simulink model "turbo_controller"  (R2025a)
settings: Solver=FixedStepAuto  StartTime=0.0  StopTime=inf  FixedStep=0.001  RelTol=1e-3
PostLoadFcn:
  | % 自动定位同目录CubeMX文件；不需要外部初始化脚本。
  | codertarget.data.setParameterValue('turbo_controller','STM32CubeMX.ProjectFile',fullfile(fileparts(get_param('turbo_controller','FileName')),'turbo_f407.ioc'));
InitFcn:
  | % 中文说明：按原控制器字段与类型创建三组接口总线；控制参数已内嵌。
  | tc_names=["EValve_Cycle" "EValve_Open" "Eblast_Cycle" "Eblast_Open" "Motor_Cycle" "Motor_Open" "EValve_Enable" "Eblast_Enable" "Motor_Enable" "SWO_Firework" "SWO_BleedAir" "EngineState" "Flag_ECUReset_Clear" "Flag_ECUReset_Save" "Flag_Reset_Enable" "Accelerator" "Nc_dem" "Nc"]; tc_types=["uint16" "uint16" "uint16" "uint16" "uint16" "uint16" "uint8" "uint8" "uint8" "uint8" "uint8" "uint8" "uint8" "uint8" "uint8" "single" "single" "single"];
  | for tc_k=1:numel(tc_names)
  |  tc_e(tc_k)=Simulink.BusElement; tc_e(tc_k).Name=char(tc_names(tc_k)); tc_e(tc_k).DataType=char(tc_types(tc_k));
  | end
  | EngineControl_Out=Simulink.Bus; EngineControl_Out.DataScope='Exported'; EngineControl_Out.Elements=tc_e;
  | clear tc_e tc_names tc_types tc_k
  | tc_names=["savedata1" "savedata2" "savedata3" "savedata4" "savedata5" "savedata6" "savedata7" "savedata8" "savedata9" "savedata10" "savedata11" "savedata12" "savedata13" "savedata14" "savedata15" "savedata16" "savedata17" "savedata18" "savedata19" "savedata20" "savedata21" "savedata22" "savedata23" "savedata24" "savedata25"]; tc_types=["single" "single" "single" "single" "single" "single" "single" "single" "single" "single" "single" "single" "single" "single" "single" "single" "single" "single" "single" "single" "single" "single" "single" "single" "single"];
  | for tc_k=1:numel(tc_names)
  |  tc_e(tc_k)=Simulink.BusElement; tc_e(tc_k).Name=char(tc_names(tc_k)); tc_e(tc_k).DataType=char(tc_types(tc_k));
  | end
  | SaveData_Out=Simulink.Bus; SaveData_Out.DataScope='Exported'; SaveData_Out.Elements=tc_e;
  | clear tc_e tc_names tc_types tc_k
  | tc_names=["senddata1" "senddata2" "senddata3" "senddata4" "senddata5" "senddata6" "senddata7" "senddata8" "senddata9" "senddata10" "senddata11" "senddata12" "senddata13" "senddata14" "senddata15" "senddata16" "senddata17" "senddata18" "senddata19" "senddata20" "senddata21" "senddata22" "senddata23" "senddata24" "senddata25" "senddata26" "senddata27" "senddata28" "senddata29"]; tc_types=["uint8" "uint8" "uint8" "uint8" "uint8" "uint8" "uint8" "uint8" "uint8" "uint8" "uint8" "uint8" "uint8" "uint8" "uint8" "uint8" "uint8" "uint8" "uint8" "uint8" "uint8" "uint8" "uint8" "uint8" "uint8" "uint8" "uint8" "uint8" "uint8"];
  | for tc_k=1:numel(tc_names)
  |  tc_e(tc_k)=Simulink.BusElement; tc_e(tc_k).Name=char(tc_names(tc_k)); tc_e(tc_k).DataType=char(tc_types(tc_k));
  | end
  | SendData_Out=Simulink.Bus; SendData_Out.DataScope='Exported'; SendData_Out.Elements=tc_e;
  | clear tc_e tc_names tc_types tc_k
  | 
  | % 以下为接口中文说明；只设置描述，不改变数值或数据类型。
  | EngineControl_Out.Description='执行控制输出（阀、电机、点火、状态及复位请求）';
  | tc_cn=["EValve_Cycle（主油阀周期计数（每计数2毫秒））" "EValve_Open（主油阀开通计数（每计数2毫秒））" "Eblast_Cycle（副油阀周期计数（每计数2毫秒））" "Eblast_Open（副油阀开通计数（每计数2毫秒））" "Motor_Cycle（起动电机周期计数）" "Motor_Open（起动电机开通计数）" "EValve_Enable（主油阀驱动使能）" "Eblast_Enable（副油阀驱动使能）" "Motor_Enable（起动电机使能）" "SWO_Firework（点火器使能（1开））" "SWO_BleedAir（引气阀使能（1开））" "EngineState（发动机状态）" "Flag_ECUReset_Clear（清除复位恢复状态请求）" "Flag_ECUReset_Save（保存复位恢复数据请求）" "Flag_Reset_Enable（处理器软件复位请求）" "Accelerator（油门／油泵给定控制量）" "Nc_dem（控制目标转速）" "Nc（发动机反馈转速（转每分））"];
  | tc_elements=EngineControl_Out.Elements;
  | for tc_k=1:numel(tc_cn)
  |  tc_elements(tc_k).Description=char(tc_cn(tc_k));
  | end
  | EngineControl_Out.Elements=tc_elements;
  | clear tc_cn tc_elements tc_k
  | SaveData_Out.Description='25项运行记录；字段含义按当前模型数据来源解释';
  | tc_cn=["savedata1（指令回显记录）" "savedata2（入口总温记录（℃））" "savedata3（电源电压记录）" "savedata4（排气温度记录（℃））" "savedata5（标定燃油压力记录）" "savedata6（副油阀占空比记录（％））" "savedata7（主油阀占空比记录（％））" "savedata8（温度修正转速记录）" "savedata9（开关输出及反馈位域）" "savedata10（物理转速记录）" "savedata11（油泵目标给定原始值）" "savedata12（起动电机占空比记录（％））" "savedata13（发动机状态码记录）" "savedata14（故障告警位域记录）" "savedata15（模型记录帧序号）" "savedata16（处理器温度记录（℃））" "savedata17（装订转速记录（沿用旧电源字段名））" "savedata18（导航高度记录）" "savedata19（飞行空速记录）" "savedata20（主阀旧记录位（恒零保留））" "savedata21（第21项保留记录（恒零））" "savedata22（保留记录项22）" "savedata23（保留记录项23）" "savedata24（保留记录项24）" "savedata25（保留记录项25）"];
  | tc_elements=SaveData_Out.Elements;
  | for tc_k=1:numel(tc_cn)
  |  tc_elements(tc_k).Description=char(tc_cn(tc_k));
  | end
  | SaveData_Out.Elements=tc_elements;
  | clear tc_cn tc_elements tc_k
  | SendData_Out.Description='29字段回传及外设命令接口；板端上位机帧只取第3至27字段';
  | tc_cn=["senddata1（回传发送允许标志（不直接上线路））" "senddata2（回传载荷长度25字节）" "senddata3（回传指令回显字节）" "senddata4（总温编码字节（℃＋80））" "senddata5（电源电压编码字节）" "senddata6（排温编码高字节）" "senddata7（排温编码低字节）" "senddata8（燃油压力编码高字节）" "senddata9（燃油压力编码低字节）" "senddata10（副油阀占空比字节（％））" "senddata11（主油阀占空比字节（％））" "senddata12（修正转速编码高字节）" "senddata13（修正转速编码低字节）" "senddata14（驱动及反馈状态位域）" "senddata15（物理转速编码高字节）" "senddata16（物理转速编码低字节）" "senddata17（油泵目标给定高字节（串口二使用））" "senddata18（油泵目标给定低字节（串口二使用））" "senddata19（起动电机占空比命令（串口一使用））" "senddata20（发动机状态码字节）" "senddata21（故障告警位域字节）" "senddata22（帧序号占位（板端另行填写））" "senddata23（处理器温度编码（℃＋50））" "senddata24（控制目标转速编码高字节）" "senddata25（控制目标转速编码低字节）" "senddata26（占位字节（板端改填实测泵速高字节））" "senddata27（占位字节（板端改填实测泵速低字节））" "senddata28（装订转速高字节（本板未发送））" "senddata29（装订转速低字节（本板未发送））"];
  | tc_elements=SendData_Out.Elements;
  | for tc_k=1:numel(tc_cn)
  |  tc_elements(tc_k).Description=char(tc_cn(tc_k));
  | end
  | SendData_Out.Elements=tc_elements;
  | clear tc_cn tc_elements tc_k
  | 
  | 
  | % FRAM模块化事务：接口类型和上电初始状态，随模型保存，无外部初始化文件。
  | clear FM_elements
  | FM_elements(1)=Simulink.BusElement;FM_elements(1).Name='phase';FM_elements(1).DataType='uint8';FM_elements(1).Dimensions=[1 1];FM_elements(1).Description='phase（当前事务阶段）';
  | FM_elements(2)=Simulink.BusElement;FM_elements(2).Name='a';FM_elements(2).DataType='uint8';FM_elements(2).Dimensions=[64 1];FM_elements(2).Description='a（启动时缓存的首区64字节）';
  | FM_elements(3)=Simulink.BusElement;FM_elements(3).Name='active';FM_elements(3).DataType='uint16';FM_elements(3).Dimensions=[1 1];FM_elements(3).Description='active（当前有效记录区地址）';
  | FM_elements(4)=Simulink.BusElement;FM_elements(4).Name='generation';FM_elements(4).DataType='uint32';FM_elements(4).Dimensions=[1 1];FM_elements(4).Description='generation（当前有效记录代号）';
  | FM_elements(5)=Simulink.BusElement;FM_elements(5).Name='record';FM_elements(5).DataType='uint8';FM_elements(5).Dimensions=[64 1];FM_elements(5).Description='record（本次冻结的待写记录）';
  | FM_elements(6)=Simulink.BusElement;FM_elements(6).Name='addr';FM_elements(6).DataType='uint16';FM_elements(6).Dimensions=[1 1];FM_elements(6).Description='addr（本次备用写入地址）';
  | FM_elements(7)=Simulink.BusElement;FM_elements(7).Name='lastSave';FM_elements(7).DataType='single';FM_elements(7).Dimensions=[1 1];FM_elements(7).Description='lastSave（上次开始保存的秒数）';
  | FM_elements(8)=Simulink.BusElement;FM_elements(8).Name='lastState';FM_elements(8).DataType='uint8';FM_elements(8).Dimensions=[1 1];FM_elements(8).Description='lastState（上次保存时的发动机状态）';
  | FM_elements(9)=Simulink.BusElement;FM_elements(9).Name='boot';FM_elements(9).DataType='boolean';FM_elements(9).Dimensions=[1 1];FM_elements(9).Description='boot（启动记录是否允许恢复）';
  | FM_elements(10)=Simulink.BusElement;FM_elements(10).Name='consumed';FM_elements(10).DataType='boolean';FM_elements(10).Dimensions=[1 1];FM_elements(10).Description='consumed（本次启动恢复通知是否已发送）';
  | FM_elements(11)=Simulink.BusElement;FM_elements(11).Name='payload';FM_elements(11).DataType='uint8';FM_elements(11).Dimensions=[20 1];FM_elements(11).Description='payload（当前20字节恢复内容）';
  | ... (+35 lines)
model workspace (MAT data in the model file):
  CRC16_Table_Reference = [0 4129 8258 12387 16516 20645 24774 28903 33032 37161 41290 45419 ... (256 elements, 256x1)]
  PE_Kaer = [0.15402 0.15402 0.12264 0.10076 0.09481 0.07601 0.07111 0.0569 0.05198 0.04926 0.05308 0.04325 ... (13 elements, 1x13)]
  PE_Nr = [21.2982 61.4260372 67.7475458 72.7394382 76.845934 80.6988798 83.8449282 86.6491912 88.9382406 89.178606 91.1938214 93.4068058 ... (13 elements, 1x13)]
  PE_Pump_Translate = 33.5999984741
  PE_RotaSpeed_Translate = 860
  PE_Taer = [0.4939154 0.4939154 0.40780982 0.34066978 0.31622756 0.30405716 0.34300244 0.26785022 0.37393554 0.23914836 0.44563948 0.31044662 ... (13 elements, 1x13)]
  PF_ACCFULLRANGE = 3360
  PF_Flag_ECUReset = 0
  PF_Flag_rx_suc = 1
  PF_Gear_Info = [40000; 45000; 50000; 55000; 57000; 59000; 60000; 61000; 61000; 61000; 61000; 61000]
  PF_K_TiaoJie = 1
  PF_Kpu = 10
  PF_MySet_Rxdata = [0 0 0 0 0 0 0 0 0 0 0 0 ... (50 elements, 50x1)]
  PF_MyUsart1_Rxdata = [0 0 0 0 0 0 0 0 0 0 0 0 ... (50 elements, 50x1)]
  PF_MyUsart2_Rxdata = [0 0 0 0 0 0 0 0 0 0 0 0 ... (50 elements, 50x1)]
  PF_Reset_Information = [0 0 0 0 0 0 0 0 0 0 0 0 ... (20 elements, 20x1)]
  PF_Sensor_X1_T4 = [0 4095]
  PF_Sensor_X2_T4 = [0 1.66666698456]
  PF_Sensor_X3_T4 = [0 504 999 1497 2010 2529 3051 3568 4076 4571 4959]
  PF_Sensor_X_P2 = [0.5 3]
  PF_Sensor_X_Poil = [0.5 3]
  PF_Sensor_X_T1t = [-50 300]
  PF_Sensor_X_Vpower = [0 3]
  PF_Sensor_X_Vpump = [0 3]
  PF_Sensor_Y1_T4 = [0 3]
  PF_Sensor_Y2_T4 = [0 5000]
  PF_Sensor_Y3_T4 = [0 100 200 300 400 500 600 700 800 900 980]
  PF_Sensor_Y_P2 = [0 1000]
  PF_Sensor_Y_Poil = [0 1000]
  PF_Sensor_Y_T1t = [-50 300]
  PF_Sensor_Y_Vpower = [0 33]
  PF_Sensor_Y_Vpump = [0 33]
  PG_CtrlMode_CloseLoop : mpt.Parameter (value not decoded)
  PG_CtrlMode_ManualAcc : mpt.Parameter (value not decoded)
  PG_CtrlMode_Origin : mpt.Parameter (value not decoded)
  PG_CtrlMode_Start : mpt.Parameter (value not decoded)
  PG_CtrlMode_Stop : mpt.Parameter (value not decoded)
  PG_ES_Clp : mpt.Parameter (value not decoded)
  PG_ES_EngStart : mpt.Parameter (value not decoded)
  PG_ES_Manual : mpt.Parameter (value not decoded)
  PG_ES_Origin : mpt.Parameter (value not decoded)
  PG_ES_Stop : mpt.Parameter (value not decoded)
  PG_Instr_BleedAirSet : mpt.Parameter (value not decoded)
  PG_Instr_CloseLoop : mpt.Parameter (value not decoded)
  PG_Instr_ECUReSet : mpt.Parameter (value not decoded)
  PG_Instr_EValveSet : mpt.Parameter (value not decoded)
  PG_Instr_EblastSet : mpt.Parameter (value not decoded)
  PG_Instr_Erase : mpt.Parameter (value not decoded)
  PG_Instr_FireWorkSet : mpt.Parameter (value not decoded)
  PG_Instr_ManualPlus : mpt.Parameter (value not decoded)
  PG_Instr_ManualrReduce : mpt.Parameter (value not decoded)
  PG_Instr_MotorSet : mpt.Parameter (value not decoded)
  PG_Instr_OilSet : mpt.Parameter (value not decoded)
  PG_Instr_SelfCheck : mpt.Parameter (value not decoded)
  PG_Instr_Start : mpt.Parameter (value not decoded)
  PG_Instr_Stop : mpt.Parameter (value not decoded)
  PG_Instr_StopZero : Simulink.Parameter (value not decoded)
  PG_Location_Air : Simulink.Parameter (value not decoded)
  PG_Location_Gnd : Simulink.Parameter (value not decoded)
  PG_ServoCtrlMode_CloseLoop : Simulink.Parameter (value not decoded)
  PG_ServoCtrlMode_CloseLoopMax : Simulink.Parameter (value not decoded)
  PG_ServoCtrlMode_CloseLoopMin : Simulink.Parameter (value not decoded)
  PG_ServoCtrlMode_ManualAcc : Simulink.Parameter (value not decoded)
  PG_ServoCtrlMode_ManualAccMax : Simulink.Parameter (value not decoded)
  PG_ServoCtrlMode_ManualAccMin : Simulink.Parameter (value not decoded)
  PG_SpeedDot_Permit : Simulink.Parameter (value not decoded)
  PL_EngineModel_Actuator = [0 10 100]
  PL_EngineModel_EngineStar_Press_P2 = [1013 1098.4 1099.144828 1099.931034 1103.613793 1162.662069 1143.793103 1131.006897 1123.186207 1117.6 1114 1111.806897 ... (127 elements, 1x127)]
  PL_EngineModel_EngineStar_RotaSpeed = [200 2000 9584 9660 10220 10240 10260 10288 10308 10368 10380 10408 ... (127 elements, 1x127)]
  PL_EngineModel_EngineStar_Temp_Exhaust = [128 129 129.1 130 131 131.1 132 133 134 134.1 135 135.1 ... (127 elements, 1x127)]
  PL_EngineModel_EngineStar_Time = [0.05 0.1 0.15 0.2 0.25 0.3 0.35 0.4 0.45 0.5 0.55 0.6 ... (127 elements, 1x127)]
  PL_EngineModel_IdleAbove_Nr = [0 21.2982 61.4260372 67.7475458 72.7394382 76.845934 80.6988798 83.8449282 86.6491912 88.9382406 89.178606 91.1938214 ... (14 elements, 1x14)]
  PL_EngineModel_IdleAbove_P2r = [0.986923266716 1.57907722675 1.81593881076 1.99358499877 2.23044658278 2.43770046879 2.65482358747 2.84233900814 3.03972366149 3.18776215149 3.25684678016 3.3950160375 ... (14 elements, 1x14)]
  PL_EngineModel_IdleAbove_Tempr = [0.0536001429337 1.07200285867 1.63301768805 1.63659103091 1.66875111667 1.72592460247 1.77595140254 1.86171163123 1.95461854565 2.03323208862 2.03323208862 2.13685903162 ... (14 elements, 1x14)]
  PL_EngineModel_IdleAbove_Ter = [0.42434128 0.42434128 0.42434128 0.30669408 0.23570008 0.22150128 0.1997974 0.23803274 0.16115638 0.24279948 0.13600422 0.31308354 ... (14 elements, 1x14)]
  PL_EngineModel_IdleAbove_Wfr = [0 10.142 23.8337 27.8905 31.9473 36.0041 40.0609 44.1177 48.1745 52.2313 52.7384 56.7952 ... (14 elements, 1x14)]
  PL_EngineModel_Press_P2 = [400 400 400 400 400 400 400 400 400 400]
  PL_EngineModel_Rotaspeed = [0 20000 96400]
  PL_EngineModel_Temp_Exhaust = [500 500 500 500 500 500 500 500 500 500]
  PL_Kaer = [0.1 0.1 0.1 0.1 0.1 0.1]
  PL_Nr = [50 60 70 80 90 100]
  PL_Taer = [0.1 0.1 0.1 0.1 0.1 0.1]
  Sig : Simulink.Signal (value not decoded)
  Ts_ms : Simulink.Parameter (value not decoded)
  false : Simulink.Parameter (value not decoded)
  true : Simulink.Parameter (value not decoded)
symbols that are objects in the model workspace (value not decoded): PG_CtrlMode_CloseLoop, PG_CtrlMode_ManualAcc, PG_CtrlMode_Origin, PG_CtrlMode_Start, PG_CtrlMode_Stop, PG_ES_Clp, PG_ES_EngStart, PG_ES_Manual, PG_ES_Origin, PG_ES_Stop, PG_Instr_BleedAirSet, PG_Instr_CloseLoop, PG_Instr_EblastSet, PG_Instr_ECUReSet, PG_Instr_Erase, PG_Instr_EValveSet, PG_Instr_FireWorkSet, PG_Instr_ManualPlus, PG_Instr_ManualrReduce, PG_Instr_MotorSet, PG_Instr_OilSet, PG_Instr_SelfCheck, PG_Instr_Start, PG_Instr_Stop, PG_Instr_StopZero, PG_ServoCtrlMode_CloseLoop, PG_ServoCtrlMode_CloseLoopMax, PG_ServoCtrlMode_CloseLoopMin, PG_ServoCtrlMode_ManualAcc, PG_ServoCtrlMode_ManualAccMax, PG_ServoCtrlMode_ManualAccMin, Ts_ms
libraries: simulink x97, stm32blockslib x10, stm32f4xxblockslib x8
(part 22 of 26)

== system turbo_controller/BoardOutput_串口封装与阀门时序/Out04_Command（电机及油泵指令）/PumpFrame（油泵指令使用原高低给定字节）_973/CRC16（只校验两个命令字节）_961/TableStep（查表更新本字节校验） ==
  note: 【中文学习说明：一次查表更新一个字节】
      | 一、输入已经是“旧CRC XOR (当前字节×256)”。
      | 输入是16位无符号整数，记作Merged（合并值）。
      |
      | 二、上路得到查表下标。
      | 合并值÷256后向下取整，取得高八位，范围0～255。
      | 这等价于参考程序中的“旧CRC高字节 XOR 当前字节”。
      | Lookup（按下标取表项）采用Zero-based（从0编号），
      | 所以0就取表的第一项，255取最后一项，不能再加1。
      |
      | 三、下路准备左移结果。
      | 先转uint32（32位无符号数），再乘256左移8位，
      | 与65535作按位AND，只保留低16位，最后转回uint16。
      | 先加宽再移位，是为了避免整数饱和破坏结果。
      | 当前字节已经在高8位，左移后移出16位范围，
      | 因此截断后与“旧CRC左移8位”的结果相同。
      |
      | 四、两路按位XOR（异或），输出更新后的16位CRC。
      | 异或的意思：两个二进制位相同得0，不同得1。
      | 本页不需要循环和记忆，输入一到就能按组合逻辑计算；
      | 跨字节的累计和每帧初值由父级CRC16模块负责。
      |
      | 五、CRC16Table（查表数据）是256项整数常量。
      | 表内容逐项复制自参考工程USER/crc.c，
      | 与NRIST_lib/NRIST_calculate.c中的表一致。
      | Selector（按下标选取）直接取一项，不做曲线插值。
      | 表中数值不是需要现场调节的控制参数。
  note: CRC16的一个字节怎样查表更新
      |
      | 父级已经把当前数据字节异或进旧CRC的高8位，形成Merged。本模块把这个16位数拆成“用哪项表”和
      | “保留哪些移位结果”两部分。
      |
      | 先取高8位：索引=floor(Merged/256)，范围0～255。用它到CRC16_Table_Reference查表；模型Select
      | or按零基索引取值，写成MATLAB数组下标时要用索引+1。
      | 另一条支路把Merged左移一个字节，即乘256，然后只保留低16位：移位值=bitand(uint32(Merged)×25
      | 6,65535)。
      |
      | 最后将表值与移位值按位异或：
      | 新CRC=bitxor(表值,移位值)。
      |
      | 例如Merged=十六进制1234，高8位12用于选表项，左移并截16位后为3400，再与表项异或。宽类型uint
      | 32是为了中间计算不先溢出，并不表示输出CRC变成32位。结果回到父级，继续处理下一个数据字节。
  Merged（旧校验值与当前字节异或后的数） : Inport  OutDataTypeStr=uint16
  CRC16Table（参考工程原始二百五十六项表） : Constant  Value=CRC16_Table_Reference  OutDataTypeStr=uint16
  Divisor（高字节换算除数） : Constant  Value=256  OutDataTypeStr=double
  Exact（转双精度做精确除法） : DataTypeConversion  OutDataTypeStr=double  SaturateOnIntegerOverflow=off  RndMeth=Floor
  HighByte（除二百五十六取高字节） : Product  Inputs=*/  OutDataTypeStr=double
  Index（向下取整得到零至二百五十五） : DataTypeConversion  OutDataTypeStr=uint32  RndMeth=Floor
  LeftByte（左移一个字节） : Product  Inputs=**  OutDataTypeStr=uint32  SaturateOnIntegerOverflow=on
  Lookup（按零基索引读取校验表） : Selector  IndexMode=Zero-based  InputPortWidth=256  IndexOptions=Index vector (port)  Indices=1  OutputSizes=1
  Mask16（保留低十六位） : Constant  Value=65535  OutDataTypeStr=uint32
  Shift16（移位结果转十六位） : DataTypeConversion  OutDataTypeStr=uint16  SaturateOnIntegerOverflow=off  RndMeth=Floor
  ShiftBase（一个字节的移位系数） : Constant  Value=256  OutDataTypeStr=uint32
  Update（查表值与移位结果异或） : simulink/Logic and Bit Operations/Bitwise Operator  logicop=XOR  UseBitMask=off  NumInputPorts=2  BitMask=bin2dec('11011001')  BitMaskRealWorld=Stored Integer
      settings: LibrarySourceBlock=|
      | hdlsllib/Logic and Bit
      | Operations/Bitwise
      | Operator
  Wide（转三十二位防止移位溢出） : DataTypeConversion  OutDataTypeStr=uint32  SaturateOnIntegerOverflow=off  RndMeth=Floor
  Wrap16（截取左移后的低十六位） : simulink/Logic and Bit Operations/Bitwise Operator  logicop=AND  UseBitMask=off  NumInputPorts=2  BitMask=bin2dec('11011001')  BitMaskRealWorld=Stored Integer
      settings: LibrarySourceBlock=|
      | hdlsllib/Logic and Bit
      | Operations/Bitwise
      | Operator
  CRC（本字节处理后的校验值） : Outport
  wires:
  Update（查表值与移位结果异或）/1 -> CRC（本字节处理后的校验值）/1
  Shift16（移位结果转十六位）/1 -> Update（查表值与移位结果异或）/2
  Lookup（按零基索引读取校验表）/1 -> Update（查表值与移位结果异或）/1
  Index（向下取整得到零至二百五十五）/1 -> Lookup（按零基索引读取校验表）/2
  CRC16Table（参考工程原始二百五十六项表）/1 -> Lookup（按零基索引读取校验表）/1
  HighByte（除二百五十六取高字节）/1 -> Index（向下取整得到零至二百五十五）/1
  Divisor（高字节换算除数）/1 -> HighByte（除二百五十六取高字节）/2
  Exact（转双精度做精确除法）/1 -> HighByte（除二百五十六取高字节）/1
  Wrap16（截取左移后的低十六位）/1 -> Shift16（移位结果转十六位）/1
  Mask16（保留低十六位）/1 -> Wrap16（截取左移后的低十六位）/2
  LeftByte（左移一个字节）/1 -> Wrap16（截取左移后的低十六位）/1
  ShiftBase（一个字节的移位系数）/1 -> LeftByte（左移一个字节）/2
  Wide（转三十二位防止移位溢出）/1 -> LeftByte（左移一个字节）/1
  Merged（旧校验值与当前字节异或后的数）/1 -> Exact（转双精度做精确除法）/1, Wide（转三十二位防止移位溢出）/1

== system turbo_controller/BoardOutput_串口封装与阀门时序/Out05_Handoff（输出交接与软件复位）/ResetService（ST官方软件复位服务）/ExecutionMode（仿真与目标运行方式）_1550/Simulation（普通仿真不复位）_1548 ==
  note: 电脑仿真时有意不执行硬件复位
      |
      | 这是ExecutionMode选中的普通仿真实现。图内为空是明确设计：STM32的NVIC_SystemReset不应在普通
      | 电脑仿真里调用。
      |
      | 外部模型仍可以计算复位请求、观察FRAM保存与控制状态，但到本分支不会真的让计算机或控制模型重
      | 新启动。要验证真实复位后的硬件启动过程，需要目标端运行，不能把空分支仿真当成已经完成硬件复
      | 位试验。

== system turbo_controller/BoardOutput_串口封装与阀门时序/Out05_Handoff（输出交接与软件复位）/ResetService（ST官方软件复位服务）/ExecutionMode（仿真与目标运行方式）_1550/Target（目标代码调用官方复位）_1549 ==
  note: 目标代码怎样执行真正的软件复位
      |
      | 本分支在STM32目标代码运行方式下使用。父级已经确认复位请求，本层官方C Caller直接调用NVIC_Sy
      | stemReset，触发控制器重新启动。
      |
      | 该服务会结束当前执行过程并从硬件启动流程重新运行，不是把EngineState改为原位的普通赋值。本
      | 层不包含FRAM保存、回读校验或串口发送完成等待；这些工作必须由外层流程安排。
      |
      | 普通电脑仿真选择另一条空实现，不执行本分支。
  NVIC_SystemReset（ST官方系统软件复位）_1547 : CCaller  FunctionName=NVIC_SystemReset

== system turbo_controller/CLM/ClpControl/Aim__Parameter_Calculate/Aim_AccMaxMin_Cal1/HoldFirst ==
  note: 进入闭环时怎样避免目标突然跳变
      |
      | 输入S_Nc_Filter是实际反馈转速，S_Dem_SpeedLoad是装订需求。两者不一定相近，如果直接把需求送
      | 误差计算，油泵给定可能出现很大瞬时变化。
      |
      | 本模块先由Hold在首次执行时记住反馈转速，外层选择支路在反馈大于0时采用锁存值，否则继续保持
      | 此前初值。记忆支路避免每次用变化中的反馈重新设起点。
      | 接着把这个起点和装订需求送M_Rate_Limiter：每次上升140、下降100，到达目标时钳住，不越过去。
      |
      | 例如起点40000、需求41000，前几次目标约为40140、40280、40420，最终停在41000；不会一开始直接
      | 跳到41000。
      | 输出再由父级加上最低40000限制，之后交闭环计算。这里限制的是目标变化，不是让传感器反馈也跟
      | 着被改写。
  S_Nc_Filter : Inport
      settings: AttributesFormatString=S_Nc_Filter（滤波后的转速）
  S_Dem_SpeedLoad : Inport  Port=2
      settings: AttributesFormatString=S_Dem_SpeedLoad（装订目标转速）
  Constant : Constant  Value=0  OutDataTypeStr=single
      settings: AttributesFormatString=Constant（常量）
  Delay : Delay  DelayLength=1
      settings: AttributesFormatString=Delay（延迟）
  Hold : Stateflow chart  Description=|  TreatAsAtomicUnit=on  RTWFcnName=Timmer  RTWFileName=EngineControl_Timmer
      | 第一次进入时只记住一次反馈转速
      | 
      | 输入Nc_First来自父级的当前滤波转速。Flag_First尚未置位时，把这个值保存到Nc_First_Hold；以后每次执行都输出保存值，不再跟着实时反馈改变。
      | 
      | 例如第一次输入40000，后续变到40500、41000，本图输出仍是40000。这样M_Rate_Limiter有稳定的起点，能够自己向装订目标推进，而不会被实时反馈不断重新拉回。
      | 
      | 这个保持只对本次图表生命周期有效；什么时候重新初始化由父级动作子系统和图表配置决定。它不会暂停模型，也不会要求转速一直保持在40000。
      settings: AttributesFormatString=Hold（保持）  RTWSystemCode=Reusable function  RTWFcnNameOpts=Use subsystem name  RTWFileNameOpts=User specified
  M_Rate_Limiter : Stateflow chart  Description=|  TreatAsAtomicUnit=on  RTWFcnName=Timmer  RTWFileName=EngineControl_Timmer
      | 目标转速怎样逐次接近装订值
      | 
      | 输入Nc_Initial是进入时锁存的反馈转速，S_Dem_SpeedLoad是上位机要求。第一次先令受限目标等于初值，再根据目标在初值上方还是下方，记住上升或下降阶段。
      | 
      | 上升时每次图表调用加140；下降时每次减100。若本次跨过装订目标，就直接取装订目标并进入跟随阶段。后续需求再次改变，仍按同样上升/下降步长逼近。
      | 可写成上升：新目标=min(旧目标+140,需求)；下降：新目标=max(旧目标-100,需求)。
      | 
      | 例如40000升到40500，输出约40140、40280、40420、40500，最后一步不是40560。每次调用的140/100是转速增量，不是每秒的变化率；按20 ms有效调用折算才有每秒意义。
      | 
      | 结果送父级形成Nc_dem，不直接改变实际转速，也不直接生成油泵给定。
      settings: AttributesFormatString=M_Rate_Limiter（中位或中间变量变化率限制器）  RTWSystemCode=Reusable function  RTWFcnNameOpts=Use subsystem name  RTWFileNameOpts=User specified
  Relational Operator : RelationalOperator  Operator=>  OutDataTypeStr=boolean  InputSameDT=off
      settings: AttributesFormatString=Relational Operator（关系比较运算）
  Switch : Switch  Criteria=u2 ~= 0  SaturateOnIntegerOverflow=off  InputSameDT=off
      settings: AttributesFormatString=Switch（开关选择）
  S_Dem_SpeedLoad_Limiter : Outport
      settings: AttributesFormatString=S_Dem_SpeedLoad_Limiter（限速率后的目标转速）
  wires:
  S_Nc_Filter/1 -> Hold/1(Nc_First), Relational Operator/1
  Switch/1 -> M_Rate_Limiter/1(Nc_Initial), Delay/1
  Constant/1 -> Relational Operator/2
  S_Dem_SpeedLoad/1 -> M_Rate_Limiter/2(S_Dem_SpeedLoad)
  M_Rate_Limiter/1(S_Dem_SpeedLoad_Limiter) -> S_Dem_SpeedLoad_Limiter/1
  Hold/1(Out) -> Switch/1
  Relational Operator/1 -> Switch/2
  Delay/1 -> Switch/3

== system turbo_controller/CLM/Manual/ManualAcc_Min_Control/手动加减/  ==
  note: 计算一次手动增减后的候选泵给定
      |
      | 以上次给定为基准：加命令输出旧值+100，减命令输出旧值-100，其他命令输出旧值。若Over_SpeedPr
      | otect为真，无论当前是否为加命令，都优先输出旧值-100。
      |
      | 例如旧值3000时，加得到3100、减得到2900，超速时也得到2900。本处只计算候选值，不负责保持窗口
      | 和最终上下限；这两项在父系统完成。100是泵给定编码的一步，不是100单位油压。
  Instr : Inport
      settings: AttributesFormatString=Instr（指令）
  Acclerator_Last : Inport  Port=2
      settings: AttributesFormatString=Acclerator_Last（油门上一周期）
  Over_SpeedProtect : Inport  Port=3
      settings: AttributesFormatString=Over_SpeedProtect（超限速度或转速保护）
  Constant2 : Constant  Value=100  OutDataTypeStr=single
      settings: AttributesFormatString=Constant2（常量2）
  N1r_idle1 : Constant  Value=PG_Instr_ManualrReduce  OutDataTypeStr=single  SampleTime=-1
      settings: AttributesFormatString=N1r_idle1（一级转速归一化值慢车1）
  N1r_idle6 : Constant  Value=PG_Instr_ManualPlus  OutDataTypeStr=single  SampleTime=-1
      settings: AttributesFormatString=N1r_idle6（一级转速归一化值慢车6）
  Relational Operator1 : RelationalOperator  Operator===  OutDataTypeStr=boolean  InputSameDT=off
      settings: AttributesFormatString=Relational Operator1（关系比较运算1）
  Relational Operator2 : RelationalOperator  Operator===  OutDataTypeStr=boolean  InputSameDT=off
      settings: AttributesFormatString=Relational Operator2（关系比较运算2）
  Sum : Sum  Inputs=|++
      settings: AttributesFormatString=Sum（加法求和）
  Sum1 : Sum  Inputs=|+-
      settings: AttributesFormatString=Sum1（加法求和1）
  Switch : Switch  Criteria=u2 ~= 0  SaturateOnIntegerOverflow=off  InputSameDT=off
      settings: AttributesFormatString=Switch（开关选择）
  Switch1 : Switch  Criteria=u2 ~= 0  SaturateOnIntegerOverflow=off  InputSameDT=off
      settings: AttributesFormatString=Switch（开关选择）
  Switch2 : Switch  Criteria=u2 ~= 0  SaturateOnIntegerOverflow=off  InputSameDT=off
      settings: AttributesFormatString=Switch（开关选择）
  Manual_Acclerator : Outport
      settings: AttributesFormatString=Manual_Acclerator（手动油门）
  wires:
  Instr/1 -> Relational Operator1/1, Relational Operator2/1
  Constant2/1 -> Sum1/2, Sum/2
  Switch2/1 -> Manual_Acclerator/1
  Acclerator_Last/1 -> Sum/1, Sum1/1, Switch/3
  Relational Operator1/1 -> Switch/2
  N1r_idle1/1 -> Relational Operator1/2
  N1r_idle6/1 -> Relational Operator2/2
  Switch/1 -> Switch1/3
  Sum/1 -> Switch1/1
  Relational Operator2/1 -> Switch1/2
  Switch1/1 -> Switch2/3
  Sum1/1 -> Switch/1, Switch2/1
  Over_SpeedProtect/1 -> Switch2/2

== system turbo_controller/COMMRead_ISM/CMMRead/T1t_P1t_Cal/Dynamic_Cal/P1H_T1H ==
  note: 按分层标准大气关系计算高度处静温和静压
      |
      | H采用km，温度采用K。11 km以下采用每升高1 km降温6.5 K的近似：
      | T1H = T10 - 6.5×H；
      | P1H = p10×(1-0.022577×H)^5.25588。
      |
      | 11 km及以上采用本模型的等温层近似：
      | T1H = T10 - 6.5×11；
      | P1H = 23.385×exp[-0.1576932×(H-11)]（kPa）。
      | 高空压力支路使用固定23.385 kPa，并不再乘参考压力p10。因此两层交界处按当前系数并非严格连续
      | ；这里如实说明现有计算，没有调整算法。
      |
      | 低层公式体现温度递减条件下的静力平衡：越高，上方空气柱越少，压力降低。高层近似温度不再下降
      | ，压力按指数衰减。标准参考T10=288.15 K、p10=101.325时，海平面输出288.15 K与101.325；11 km
      | 处温度216.65 K。
      |
      | 这是高度大气近似，不包含天气、湿度和进气损失。当前没有由此自动识别超出适用高度范围的传感器
      | 故障。
  H : Inport
      settings: AttributesFormatString=H（高度）
  T10 : Inport  Port=2
      settings: AttributesFormatString=T10（入口参考温度）
  p10 : Inport  Port=3
      settings: AttributesFormatString=p10（压力或比例变量10）
  Constant1 : Constant  Value=6.5
      settings: AttributesFormatString=Constant1（常量1）
  Constant10 : Constant  Value=11
      settings: AttributesFormatString=Constant10（常量10）
  Constant11 : Constant  Value=11
      settings: AttributesFormatString=Constant11（常量11）
  Constant12 : Constant  Value=-0.1576932
      settings: AttributesFormatString=Constant12（常量12）
  Constant3 : Constant
      settings: AttributesFormatString=Constant3（常量3）
  Constant4 : Constant  Value=0.022577
      settings: AttributesFormatString=Constant4（常量4）
  Constant5 : Constant  Value=23.385
      settings: AttributesFormatString=Constant5（常量5）
  Constant6 : Constant  Value=5.25588
      settings: AttributesFormatString=Constant6（常量6）
  Constant7 : Constant  Value=11
      settings: AttributesFormatString=Constant7（常量7）
  Constant8 : Constant  Value=6.5
      settings: AttributesFormatString=Constant8（常量8）
  Data Type Conversion1 : DataTypeConversion  OutDataTypeStr=single  SaturateOnIntegerOverflow=off  RndMeth=Floor
      settings: AttributesFormatString=Data Type Conversion1（数据类型转换1）
  Data Type Conversion5 : DataTypeConversion  OutDataTypeStr=single  SaturateOnIntegerOverflow=off  RndMeth=Floor
      settings: AttributesFormatString=Data Type Conversion5（数据类型转换5）
  Math Function : Math  Operator=pow  SignedPower=on
      settings: AttributesFormatString=Math Function（数学函数）
  Math Function1 : Math  SignedPower=on
      settings: AttributesFormatString=Math Function1（数学函数1）
  Product{,1..5} (6 alike) : Product
      Product settings: AttributesFormatString=Product（乘法）
      Product1 settings: AttributesFormatString=Product1（乘法1）
      Product2 settings: AttributesFormatString=Product2（乘法2）
      Product3 settings: AttributesFormatString=Product3（乘法3）
      Product4 settings: AttributesFormatString=Product4（乘法4）
      Product5 settings: AttributesFormatString=Product5（乘法5）
  Relational Operator : RelationalOperator  Operator=<  OutDataTypeStr=boolean  InputSameDT=off
      settings: AttributesFormatString=Relational Operator（关系比较运算）
  Sum{,2..4} (4 alike) : Sum  Inputs=|+-
      Sum settings: AttributesFormatString=Sum（加法求和）
      Sum2 settings: AttributesFormatString=Sum2（加法求和2）
      Sum3 settings: AttributesFormatString=Sum3（加法求和3）
      Sum4 settings: AttributesFormatString=Sum4（加法求和4）
  Switch : Switch  Criteria=u2 ~= 0  SaturateOnIntegerOverflow=off  InputSameDT=off
      settings: AttributesFormatString=Switch（开关选择）
  Switch1 : Switch  Criteria=u2 ~= 0  SaturateOnIntegerOverflow=off  InputSameDT=off
      settings: AttributesFormatString=Switch（开关选择）
  T1H : Outport
      settings: AttributesFormatString=T1H（对应高度的入口温度）
  P1H : Outport  Port=2
      settings: AttributesFormatString=P1H（对应高度的入口压力）
  wires:
  Constant1/1 -> Product/2
  Product/1 -> Sum/2
  p10/1 -> Product1/1
  Constant3/1 -> Sum2/1
  H/1 -> [H_km]
  [H_km] -> Product/1
  [H_km] -> Product2/2, Sum3/1
  Constant4/1 -> Product2/1
  Product2/1 -> Sum2/2
  Sum2/1 -> Math Function/1
  Constant6/1 -> Math Function/2
  Math Function/1 -> Product1/2
  [H_km] -> Relational Operator/1
  Constant7/1 -> Relational Operator/2
  Switch/1 -> Data Type Conversion5/1
  Constant8/1 -> Product3/2
  T10/1 -> Sum4/1, Sum/1
  Product3/1 -> Sum4/2
  Constant10/1 -> Product3/1
  Switch1/1 -> Data Type Conversion1/1
  Constant5/1 -> Product4/1
  Math Function1/1 -> Product4/2  "高空指数压比"
  Constant11/1 -> Sum3/2
  Product5/1 -> Math Function1/1
  Sum3/1 -> Product5/1
  Constant12/1 -> Product5/2
  Data Type Conversion5/1 -> T1H/1
  Data Type Conversion1/1 -> P1H/1
  Sum4/1 -> Switch/3  "高空静温（K）"
  Sum/1 -> Switch/1  "低空静温（K）"
  Product4/1 -> Switch1/3  "高空静压（kPa）"
  Product1/1 -> Switch1/1  "低空静压（kPa）"
  Relational Operator/1 -> Switch1/2, Switch/2

== system turbo_controller/COMMRead_ISM/CMMRead/T1t_P1t_Cal/Dynamic_Cal/dynamic  ==
  note: 把飞行空速对应的动能计入进气总温、总压
      |
      | 输入静温T1H（K）、静压P1H和空速V=AirSpeed（m/s）。先求当地声速，再求马赫数：
      | a = sqrt(1.4×287.06×T1H)；
      | M = V/a。
      | 1.4为空气比热比，287.06是空气气体常数，a的单位m/s。M表示飞行速度是当地声速的多少倍，不是把
      | 空速直接除以固定340。
      |
      | 再计算理想气流减速后的总量：
      | 温升因子 = 1+0.2×M²；
      | T1t = T1H×温升因子；
      | P1t = P1H×温升因子^3.5。
      | 3.5=1.4/0.4，模型恢复系数当前为1。
      |
      | 例如静温288.15 K时声速约340.3 m/s，空速100 m/s得到M约0.294，温升因子约1.0173，总温约293.13
      |  K；总压约为静压的1.0616倍。空速0时总温、总压回到静温、静压。
      |
      | 公式假设理想气体和等熵减速，没有额外模拟进气道摩擦、激波或测量误差。压力单位沿用输入，不能
      | 因为计算名称含dynamic就把结果当成单独的动压。
  T1H : Inport
      settings: AttributesFormatString=T1H（对应高度的入口温度）
  P1H : Inport  Port=2
      settings: AttributesFormatString=P1H（对应高度的入口压力）
  AirSpeed : Inport  Port=3
      settings: AttributesFormatString=AirSpeed（空速）
  Constant1 : Constant  Value=0.2
      settings: AttributesFormatString=Constant1（常量1）
  Constant2 : Constant  Value=1.4
      settings: AttributesFormatString=Constant2（常量2）
  Constant3 : Constant  Value=0.4
      settings: AttributesFormatString=Constant3（常量3）
  Constant7 : Constant
      settings: AttributesFormatString=Constant7（常量7）
  Divide : Product  Inputs=*/
      settings: AttributesFormatString=Divide（除法）
  HuiFuXiShu : Constant
      settings: AttributesFormatString=HuiFuXiShu（恢复系数）
  Math Function : Math  Operator=square  SignedPower=on
      settings: AttributesFormatString=Math Function（数学函数）
  Math Function1 : Math  Operator=pow  SignedPower=on
      settings: AttributesFormatString=Math Function1（数学函数1）
  Product{,1..3} (4 alike) : Product
      Product settings: AttributesFormatString=Product（乘法）
      Product1 settings: AttributesFormatString=Product1（乘法1）
      Product2 settings: AttributesFormatString=Product2（乘法2）
      Product3 settings: AttributesFormatString=Product3（乘法3）
  Product4 : Product  Inputs=*/
      settings: AttributesFormatString=Product4（乘法4）
  Product5 : Product  Inputs=***
      settings: AttributesFormatString=Product5（乘法5）
  Sqrt : Sqrt
      settings: AttributesFormatString=Sqrt（平方根）
  Sum : Sum  Inputs=|++
      settings: AttributesFormatString=Sum（加法求和）
  constant5 : Constant  Value=single(1.4)  OutDataTypeStr=single  SampleTime=-1
      settings: AttributesFormatString=constant5（常量5）
  constant6 : Constant  Value=single(287.06)  OutDataTypeStr=single  SampleTime=-1
      settings: AttributesFormatString=constant6（常量6）
  T1t : Outport
      settings: AttributesFormatString=T1t（入口总温）
  P1t : Outport  Port=2
      settings: AttributesFormatString=P1t（入口总压）
  wires:
  Product/1 -> T1t/1
  Constant7/1 -> Sum/1
  Product1/1 -> Sum/2
  Sum/1 -> Product/2, Math Function1/1  "总温比 τ"
  Constant1/1 -> Product1/1
  AirSpeed/1 -> Product4/1
  [Ma] -> Math Function/1
  Math Function/1 -> Product1/2  "马赫数平方 M²"
  Constant2/1 -> Divide/1
  Constant3/1 -> Divide/2
  Divide/1 -> Math Function1/2  "等熵压力指数 3.5"
  Math Function1/1 -> Product2/1  "理想总压比 π"
  P1H/1 -> Product2/2
  Product2/1 -> Product3/1
  HuiFuXiShu/1 -> Product3/2
  Product3/1 -> P1t/1
  constant6/1 -> Product5/3
  constant5/1 -> Product5/2
  T1H/1 -> Product5/1, Product/1
  Sqrt/1 -> Product4/2  "当地声速 a（m/s）"
  Product5/1 -> Sqrt/1
  Product4/1 -> [Ma]  "飞行马赫数 M"

== system turbo_controller/COMMRead_ISM/ISM/AnalogFilter_Nc/GeneralFilter/Subsystem ==
  note: 对经过有效性判断的转速做一阶低通，减小采样抖动
      |
      | 每次把本拍输入与上次滤波结果按比例相加：
      | 本拍输出=α×本拍输入+β×上次输出；
      | α=Ts/(T+Ts)，β=T/(T+Ts)。
      |
      | 当前T=0.067 s，Ts=Ts_ms/1000=0.02 s，因此α约0.229885、β约0.770115。新输入约占23%，旧结果
      | 约占77%。例如上次输出100、本次输入200，本次滤波结果约123，随后逐步靠近200。
      |
      | 它抑制快速波动，也会让真实变化稍有滞后；不负责把ADC计数变成物理量，也不单凭滤波判定传感器
      | 故障。输出送Nc_Filter，参与控制与故障处理。
  In1 : Inport
  Constant1 : Constant  Value=Ts_ms  OutDataTypeStr=single  SampleTime=-1
      settings: AttributesFormatString=Constant1（常量1）
  Constant2 : Constant  Value=1000  OutDataTypeStr=single  SampleTime=-1
      settings: AttributesFormatString=Constant2（常量2）
  Constant6 : Constant  Value=single(0.067)  OutDataTypeStr=single  SampleTime=-1
      settings: AttributesFormatString=Constant6（常量6）
  Divide : Product  Inputs=*/
      settings: AttributesFormatString=Divide（除法）
  Integer Delay1 : Delay  DelayLength=1  InitialCondition=0
      settings: AttributesFormatString=Integer Delay1（整数延迟1）
  Product2 : Product  RndMeth=Zero
      settings: AttributesFormatString=Product2（乘法2）
  Product3 : Product  RndMeth=Zero
      settings: AttributesFormatString=Product3（乘法3）
  Subsystem1 : Subsystem  Description=|
      | 计算低通滤波中新样本的权重
      | 
      | 输入T为滤波时间常数（s），T_Sampling为采样周期（s）。输出α=T_Sampling/(T+T_Sampling)，供父级乘以本拍的新输入。
      | 
      | 当前T=0.067、采样周期0.02，α=0.02/0.087≈0.229885。也就是每拍只采用约23%的新值，另外约77%由历史结果补足。时间常数越大，新值权重越小，结果越平稳但响应越慢。
      | 
      | 本模块只算一个无量纲系数，不含延迟，也不直接输出温度、压力或转速。两项时间输入必须使用同一单位。
      settings: AttributesFormatString=Subsystem1（子系统1）
      mask Display: disp('T_S\n---------------\nT_S + T')
  Subsystem2 : Subsystem  Description=|
      | 计算低通滤波中历史结果的权重
      | 
      | 输入T为时间常数，T_Sampling为采样周期，两者都用s。输出β=T/(T+T_Sampling)，供父级乘以上一次滤波结果。
      | 
      | 当前T=0.067、采样周期0.02，β≈0.770115；与另一支路新样本权重α≈0.229885相加为1。这样常值输入最终会稳定在原值，不会因为反复相加而不断放大。
      | 
      | 本模块只计算系数，历史结果由父级延迟块保存。若把20 ms误传成20 s，权重和滤波速度都会完全改变，因此父级先将Ts_ms除以1000。
      settings: AttributesFormatString=Subsystem2（子系统2）
      mask Display: disp('T\n---------------\nT_S + T')
  Sum3 : Sum  Inputs=|++
      settings: AttributesFormatString=Sum3（加法求和3）
  Out1 : Outport
  wires:
  Sum3/1 -> Out1/1, Integer Delay1/1
  Divide/1 -> Subsystem2/2(T_Sampling), Subsystem1/2(T_Sampling)  "T_S（采样周期）"
  Product3/1 -> Sum3/2
  Constant2/1 -> Divide/2
  Product2/1 -> Sum3/1
  Subsystem2/1(Out) -> Product3/2
  Constant6/1 -> Subsystem2/1(T), Subsystem1/1(T)  "T（滤波时间常数）"
  Integer Delay1/1 -> Product3/1
  Constant1/1 -> Divide/1
  Subsystem1/1(Out) -> Product2/2
  In1/1 -> Product2/1

== system turbo_controller/BoardInput_输入换算与协议解析/In01_Host（上位机命令解析）/Receive（逐字节组帧与保持有效结果）_108/Step02_拼帧并记住未收完的数据/Collect（帧头识别与缓存推进）_66/Step01_判断收帧阶段与AA55 ==
  note: 第一步：看现在收到哪里，并识别AA、55
      |
      | 只看Position和Byte，不修改缓存，不保存历史。输出三个判断：是否正在找第一个AA、当前字节是否
      | AA、是否发生第二帧头不匹配。
      |
      | Position=0：还没确认帧头，正在找AA。
      | Position=1：已经见到AA，期望下一个是55。
      | Position≥2：头部已确认，后续字节属于帧内数据。
      |
      | AA是十六进制，十进制为170；55是十六进制，十进制为85。判断式：
      | 等待AA=(Position==0)；
      | 字节是AA=(Byte==170)；
      | 第二帧头错=(Position==1) AND (Byte!=85)。
      |
      | 例：Position=1、Byte=AA时，字节是AA和第二帧头错都为真。这并不冲突：它表示没等到55，但可以
      | 把这个AA视作重新找头的机会。是否写入、位置如何调整由后面两步分别处理。
      |
      | 本步骤不检查Active；本字节无效时，后面的写入和位置保持分支会阻止它改变状态。
  输入1_本项字节 : Inport
  输入2_本次之前已收字节数 : Inport  Port=2
  位置为0_等待AA : RelationalOperator  Operator===  OutDataTypeStr=boolean  RndMeth=Simplest  InputSameDT=off
  位置为1_等待55 : RelationalOperator  Operator===  OutDataTypeStr=boolean  RndMeth=Simplest  InputSameDT=off
  已见AA时位置1 : Constant  OutDataTypeStr=uint16
  帧头55_十进制85 : Constant  Value=85  OutDataTypeStr=uint8
  帧头AA_十进制170 : Constant  Value=170  OutDataTypeStr=uint8
  当前字节不是55 : RelationalOperator  Operator=~=  OutDataTypeStr=boolean  RndMeth=Simplest  InputSameDT=off
  当前字节是否AA : RelationalOperator  Operator===  OutDataTypeStr=boolean  RndMeth=Simplest  InputSameDT=off
  等待55却收到其他值 : Logic  IconShape=distinctive  AllPortsSameDT=off  OutDataTypeStr=boolean
  起始位置0 : Constant  Value=0  OutDataTypeStr=uint16
  输出1_当前字节等于AA : Outport
  输出2_正在寻找第一个AA : Outport  Port=2
  输出3_第二帧头不匹配 : Outport  Port=3
  wires:
  等待55却收到其他值/1 -> 输出3_第二帧头不匹配/1
  位置为0_等待AA/1 -> 输出2_正在寻找第一个AA/1
  当前字节是否AA/1 -> 输出1_当前字节等于AA/1
  起始位置0/1 -> 位置为0_等待AA/2
  已见AA时位置1/1 -> 位置为1_等待55/2
  输入2_本次之前已收字节数/1 -> 位置为1_等待55/1, 位置为0_等待AA/1
  帧头55_十进制85/1 -> 当前字节不是55/2
  帧头AA_十进制170/1 -> 当前字节是否AA/2
  输入1_本项字节/1 -> 当前字节是否AA/1, 当前字节不是55/1
  当前字节不是55/1 -> 等待55却收到其他值/2
  位置为1_等待55/1 -> 等待55却收到其他值/1

== system turbo_controller/BoardInput_输入换算与协议解析/In01_Host（上位机命令解析）/Receive（逐字节组帧与保持有效结果）_108/Step02_拼帧并记住未收完的数据/Collect（帧头识别与缓存推进）_66/Step02_判断本字节能否写入 ==
  note: 第二步：决定本字节是否允许写进帧缓存
      |
      | 收帧必须先找到头，所以不是每个字节都写。将第一步的三个判断与Active组合：
      |
      | 允许写入=Active AND [
      |   (正在等AA AND 字节是AA)
      |   OR (不在等AA AND 第二帧头没有错)
      | ]。
      |
      | 分别理解：
      | 还在找AA时，只写AA，其他噪声不进入缓存；
      | 已经见到AA、等待55时，只写正确的55；
      | 头部已经确认后，按顺序接收普通数据，不因数据恰好是AA/55就重新找头；
      | Active为假时，上述条件再合适也不写。
      |
      | 例：已见AA后又来AA，本步骤不把第二个AA写进第2项；后面的重同步位置逻辑仍保留“已见AA”的状
      | 态，继续等55。
      |
      | 输出只是一项布尔写许可，送第四步。它不产生新缓存，也不判断整帧校验。
  输入1_正在寻找第一个AA : Inport
  输入2_当前字节等于AA : Inport  Port=2
  输入3_第二帧头不匹配 : Inport  Port=3
  输入4_本项字节有效 : Inport  Port=4
  字节符合收帧规则 : Logic  Operator=OR  IconShape=distinctive  AllPortsSameDT=off  OutDataTypeStr=boolean
  已经越过寻找AA阶段 : Logic  Operator=NOT  Inputs=1  IconShape=distinctive  AllPortsSameDT=off  OutDataTypeStr=boolean
  已过起点且第二帧头没错 : Logic  IconShape=distinctive  AllPortsSameDT=off  OutDataTypeStr=boolean
  本字节有效且允许写入 : Logic  IconShape=distinctive  AllPortsSameDT=off  OutDataTypeStr=boolean
  第二帧头没有错 : Logic  Operator=NOT  Inputs=1  IconShape=distinctive  AllPortsSameDT=off  OutDataTypeStr=boolean
  起点遇到AA : Logic  IconShape=distinctive  AllPortsSameDT=off  OutDataTypeStr=boolean
  输出1_本字节允许写缓存 : Outport
  wires:
  本字节有效且允许写入/1 -> 输出1_本字节允许写缓存/1
  字节符合收帧规则/1 -> 本字节有效且允许写入/2
  输入4_本项字节有效/1 -> 本字节有效且允许写入/1
  输入3_第二帧头不匹配/1 -> 第二帧头没有错/1
  已过起点且第二帧头没错/1 -> 字节符合收帧规则/2
  起点遇到AA/1 -> 字节符合收帧规则/1
  第二帧头没有错/1 -> 已过起点且第二帧头没错/2
  已经越过寻找AA阶段/1 -> 已过起点且第二帧头没错/1
  输入2_当前字节等于AA/1 -> 起点遇到AA/2
  输入1_正在寻找第一个AA/1 -> 起点遇到AA/1, 已经越过寻找AA阶段/1

== system turbo_controller/BoardInput_输入换算与协议解析/In01_Host（上位机命令解析）/Receive（逐字节组帧与保持有效结果）_108/Step02_拼帧并记住未收完的数据/Collect（帧头识别与缓存推进）_66/Step03_计算写入位置与是否满帧 ==
  note: 第三步：算本次写到第几项，并判断是否到帧尾
      |
      | Position表示本次之前已接收多少项。本次候选写入位置=Position+1；帧长度固定为14，达到帧尾=(
      | 候选写入位置==14)。
      |
      | 例如Position=0时，候选位置是1，AA应写到第1项；Position=1时，55应写到第2项；Position=13时，
      | 本次候选位置是14，这是最后一项。
      |
      | 注意这里算的是“候选位置”：即使Active为假，仍可计算Position+1，但第四、第五步会保持缓存和
      | 位置。不能仅因候选位置等于14就认定收到新帧。
      |
      | 候选位置送第四步写缓存；它及“达到帧尾”标志也送第五步，决定继续推进还是收齐后回0。本处不
      | 保存Position，也不清空缓存。
  输入1_本次之前已收字节数 : Inport
  候选位置是否到帧尾 : RelationalOperator  Operator===  OutDataTypeStr=boolean  RndMeth=Simplest  InputSameDT=off
  固定帧长14 : Constant  Value=14  OutDataTypeStr=uint16
  本次候选位置加一 : Sum  SaturateOnIntegerOverflow=on  OutDataTypeStr=Inherit: Same as first input
  每次推进1项 : Constant  OutDataTypeStr=uint16
  输出1_候选位置达到帧长 : Outport
  输出2_候选写入位置 : Outport  Port=2
  wires:
  候选位置是否到帧尾/1 -> 输出1_候选位置达到帧长/1
  每次推进1项/1 -> 本次候选位置加一/2
  输入1_本次之前已收字节数/1 -> 本次候选位置加一/1
  固定帧长14/1 -> 候选位置是否到帧尾/2
  本次候选位置加一/1 -> 候选位置是否到帧尾/1, 输出2_候选写入位置/1

== system turbo_controller/BoardInput_输入换算与协议解析/In01_Host（上位机命令解析）/Receive（逐字节组帧与保持有效结果）_108/Step02_拼帧并记住未收完的数据/Collect（帧头识别与缓存推进）_66/Step04_写入字节或保持原缓存 ==
  note: 第四步：只更新应写的一项，其他内容保留
      |
      | 输入包括旧缓存、本次Byte、候选写入位置和写许可。先将索引取min(候选位置,14)，防止索引超过14
      | 项缓存上界，再用Assignment生成“把这一项换成Byte”的候选数组。
      |
      | 最终选择：写许可为真输出更新数组；写许可为假直接输出旧缓存。即使内部算出了候选更新，只要没
      | 有许可，它也不会成为输出。
      |
      | 例：旧位置为5，本次允许接收，就把第6项换成本字节，其他13项保持；若本字节无效或第二帧头错，
      | 整份缓存保持。缓存里旧的尾部数据并不会每次清零，所以必须配合Complete和后续校验使用，不能只
      | 看数组里有值就当作新帧。
      |
      | 本步骤不保存跨调用记忆。输出回外层的缓存记忆，供下一个字节/下一批数据继续使用。位置更新与
      | 收齐事件在第五步处理。
  输入1_本字节允许写缓存 : Inport
  输入2_上一份候选缓存 : Inport  Port=2
  输入3_候选写入位置 : Inport  Port=3
  输入4_本项字节 : Inport  Port=4
  不允许写则沿用旧缓存 : Switch  Criteria=u2 ~= 0  SaturateOnIntegerOverflow=off  InputSameDT=off
  只替换缓存这一项 : Assignment  DiagnosticForDimensions=Warning  IndexOptions=Index vector (port)  Indices=1  OutputSizes=1
  索引不超过14 : MinMax  Inputs=2
  缓存最大索引14 : Constant  Value=14  OutDataTypeStr=uint16
  输出1_更新后的候选缓存 : Outport
  wires:
  不允许写则沿用旧缓存/1 -> 输出1_更新后的候选缓存/1
  索引不超过14/1 -> 只替换缓存这一项/3
  输入4_本项字节/1 -> 只替换缓存这一项/2
  缓存最大索引14/1 -> 索引不超过14/2
  输入3_候选写入位置/1 -> 索引不超过14/1
  输入2_上一份候选缓存/1 -> 只替换缓存这一项/1, 不允许写则沿用旧缓存/3
  输入1_本字节允许写缓存/1 -> 不允许写则沿用旧缓存/2
  只替换缓存这一项/1 -> 不允许写则沿用旧缓存/1

== system turbo_controller/BoardInput_输入换算与协议解析/In01_Host（上位机命令解析）/Receive（逐字节组帧与保持有效结果）_108/Step02_拼帧并记住未收完的数据/Collect（帧头识别与缓存推进）_66/Step05_更新收帧位置并报告收齐 ==
  note: 第五步：确定下一次收帧位置，并报告刚收齐
      |
      | 先按收帧阶段选择下一Position：
      | 正在找AA：本字节是AA则到1，否则到0；
      | 正在等55但本字节不匹配：若又是AA则保持1，其他值回0；
      | 正常收数据：未到帧尾就采用Position+1，达到14项后回0，准备找下一帧头。
      | 最后再检查Active：为假时直接保留旧Position，上面的候选变化都不采用。
      |
      | 收齐事件=Active AND 不在等待第一个AA AND 第二帧头没错 AND 达到14项。
      | 因此它只在有效字节刚补上最后一项时为真，不是缓存里有14项就一直为真。位置回0时，完整缓存仍
      | 保留供外层校验。
      |
      | 例：Position=13，有效字节到来，输出Position=0且Complete=true；同样的位置但Active=false，则
      | 输出仍为13且Complete=false。AA、AA、55的序列依次得到位置1、1、2。
      |
      | 本页不验证CRC或累加/异或校验，也不等待下一个20 ms节拍；Complete交外层决定是否接受这条候选
      | 帧。
  输入1_当前字节等于AA : Inport
  输入2_本项字节有效 : Inport  Port=2
  输入3_候选位置达到帧长 : Inport  Port=3
  输入4_候选写入位置 : Inport  Port=4
  输入5_本次之前已收字节数 : Inport  Port=5
  输入6_正在寻找第一个AA : Inport  Port=6
  输入7_第二帧头不匹配 : Inport  Port=7
  AA匹配结果转成0或1 : DataTypeConversion  OutDataTypeStr=uint16  RndMeth=Round
  刚收齐一帧 : Logic  Inputs=4  IconShape=distinctive  AllPortsSameDT=off  OutDataTypeStr=boolean
  已经越过寻找AA阶段 : Logic  Operator=NOT  Inputs=1  IconShape=distinctive  AllPortsSameDT=off  OutDataTypeStr=boolean
  无效字节保持原位置 : Switch  Criteria=u2 ~= 0  SaturateOnIntegerOverflow=off  InputSameDT=off
  满帧回0_未满继续 : Switch  Criteria=u2 ~= 0  SaturateOnIntegerOverflow=off  InputSameDT=off
  第二帧头没有错 : Logic  Operator=NOT  Inputs=1  IconShape=distinctive  AllPortsSameDT=off  OutDataTypeStr=boolean
  第二帧头错则重新找 : Switch  Criteria=u2 ~= 0  SaturateOnIntegerOverflow=off  InputSameDT=off
  起始位置0 : Constant  Value=0  OutDataTypeStr=uint16
  起点只接收AA : Switch  Criteria=u2 ~= 0  SaturateOnIntegerOverflow=off  InputSameDT=off
  输出1_下一次已收字节数 : Outport
  输出2_本字节刚收齐 : Outport  Port=2
  wires:
  刚收齐一帧/1 -> 输出2_本字节刚收齐/1
  无效字节保持原位置/1 -> 输出1_下一次已收字节数/1
  第二帧头错则重新找/1 -> 起点只接收AA/3
  满帧回0_未满继续/1 -> 第二帧头错则重新找/3
  AA匹配结果转成0或1/1 -> 第二帧头错则重新找/1, 起点只接收AA/1
  输入7_第二帧头不匹配/1 -> 第二帧头没有错/1, 第二帧头错则重新找/2
  输入6_正在寻找第一个AA/1 -> 已经越过寻找AA阶段/1, 起点只接收AA/2
  输入5_本次之前已收字节数/1 -> 无效字节保持原位置/3
  起点只接收AA/1 -> 无效字节保持原位置/1
  输入4_候选写入位置/1 -> 满帧回0_未满继续/3
  起始位置0/1 -> 满帧回0_未满继续/1
  输入3_候选位置达到帧长/1 -> 满帧回0_未满继续/2, 刚收齐一帧/4
  第二帧头没有错/1 -> 刚收齐一帧/3
  已经越过寻找AA阶段/1 -> 刚收齐一帧/2
  输入2_本项字节有效/1 -> 无效字节保持原位置/2, 刚收齐一帧/1
  输入1_当前字节等于AA/1 -> AA匹配结果转成0或1/1

== system turbo_controller/BoardInput_输入换算与协议解析/In01_Host（上位机命令解析）/Receive（逐字节组帧与保持有效结果）_108/Step03_检查完整性与双校验/Verify（完整帧校验）_93/Checksum（累加与异或校验）_85 ==
  note: 一段字节怎样得到累加和异或两种校验
      |
      | 输入是一整段需要校验的字节。每帧开始，两路累积值都从0开始；For Iterator按顺序取出每个字节
      | ，同时更新两路结果。
      |
      | 累加这一路只保留低8位：
      | 新累加值 = mod(旧累加值 + 当前字节,256)。
      | 例如三个字节为200、100、1，总和301，最后校验字节为45，不让普通uint8溢出替代明确的取余规则
      | 。
      |
      | 异或这一路逐位计算：
      | 新异或值 = bitxor(旧异或值,当前字节)。
      | 相同比特异或得到0，不同比特得到1。它与“所有数相加”是两种不同检查。
      |
      | 接收侧拿这两个结果和帧尾比较，发送侧把结果追加到帧尾。父级负责规定哪些字节参加计算；本模块
      | 不验证帧头，也不能替换电机/油泵协议使用的CRC16。
  Bytes（待校验字节）_71 : Inport  OutDataTypeStr=uint8
  Add（加减运算）_78 : Sum  SaturateOnIntegerOverflow=on  OutDataTypeStr=Inherit: Same as first input
  Cast（数据类型转换）_76 : DataTypeConversion  OutDataTypeStr=double  RndMeth=Round
  Cast（数据类型转换）_77 : DataTypeConversion  OutDataTypeStr=double  RndMeth=Round
  Cast（数据类型转换）_81 : DataTypeConversion  OutDataTypeStr=uint8  RndMeth=Floor
  Constant（常量）_79 : Constant  Value=256  OutDataTypeStr=double
  EachByte（逐字节累加与异或）_72 : ForIterator  ResetStates=reset  IterationLimit=12  IterationVariableDataType=uint32
  Select（按索引取元素）_75 : Selector  InputPortWidth=12  IndexOptions=Index vector (port)  Indices=1  OutputSizes=1
  Store_uint8（按八位无符号数保存状态）_536558 : DataTypeConversion  Description=为反馈回路显式指定原程序的状态类型，保持原状态更新节拍。  OutDataTypeStr=uint8  RndMeth=Round
  Sum（本帧累加器）_73 : UnitDelay  InitialCondition=uint8(0)  SampleTime=-1  HasFrameUpgradeWarning=on
  Wrap8（累加后只保留八位）_80 : Math  Operator=mod
  XorStep（异或一个字节）_82 : simulink/Logic and Bit Operations/Bitwise Operator  logicop=XOR  UseBitMask=off  NumInputPorts=2  BitMask=bin2dec('11011001')  BitMaskRealWorld=Stored Integer
      settings: LibrarySourceBlock=|
      | hdlsllib/Logic and Bit
      | Operations/Bitwise
      | Operator
  Xor（本帧异或器）_74 : UnitDelay  InitialCondition=uint8(0)  SampleTime=-1  HasFrameUpgradeWarning=on
  Sum8（八位累加结果）_83 : Outport
  Xor8（八位异或结果）_84 : Outport  Port=2
  wires:
  XorStep（异或一个字节）_82/1 -> Xor8（八位异或结果）_84/1, Store_uint8（按八位无符号数保存状态）_536558/1  "XorStep（异或一个字节）"
  Xor（本帧异或器）_74/1 -> XorStep（异或一个字节）_82/1  "Xor（本帧异或器）"
  Select（按索引取元素）_75/1 -> XorStep（异或一个字节）_82/2, Cast（数据类型转换）_77/1  "Select（按索引取元素）"
  Store_uint8（按八位无符号数保存状态）_536558/1 -> Xor（本帧异或器）_74/1
  Bytes（待校验字节）_71/1 -> Select（按索引取元素）_75/1  "Bytes（待校验字节）"
  EachByte（逐字节累加与异或）_72/1 -> Select（按索引取元素）_75/2  "EachByte（逐字节累加与异或）"
  Sum（本帧累加器）_73/1 -> Cast（数据类型转换）_76/1  "Sum（本帧累加器）"
  Cast（数据类型转换）_76/1 -> Add（加减运算）_78/1  "Cast（数据类型转换）"
  Cast（数据类型转换）_77/1 -> Add（加减运算）_78/2  "Cast（数据类型转换）"
  Add（加减运算）_78/1 -> Wrap8（累加后只保留八位）_80/1  "Add（加减运算）"
  Constant（常量）_79/1 -> Wrap8（累加后只保留八位）_80/2  "Constant（常量）"
  Wrap8（累加后只保留八位）_80/1 -> Cast（数据类型转换）_81/1  "Wrap8（累加后只保留八位）"
  Cast（数据类型转换）_81/1 -> Sum8（八位累加结果）_83/1, Sum（本帧累加器）_73/1  "Cast（数据类型转换）"

== system turbo_controller/BoardInput_输入换算与协议解析/In02_Motor（电机反馈解析）/Receive（逐字节组帧与保持有效结果）_235/Step02_拼帧并保存半帧/Collect（帧头识别与缓存推进）_167/Step01_判断收帧阶段与AA55 ==
  note: 第一步：看现在收到哪里，并识别AA、55
      |
      | 只看Position和Byte，不修改缓存，不保存历史。输出三个判断：是否正在找第一个AA、当前字节是否
      | AA、是否发生第二帧头不匹配。
      |
      | Position=0：还没确认帧头，正在找AA。
      | Position=1：已经见到AA，期望下一个是55。
      | Position≥2：头部已确认，后续字节属于帧内数据。
      |
      | AA是十六进制，十进制为170；55是十六进制，十进制为85。判断式：
      | 等待AA=(Position==0)；
      | 字节是AA=(Byte==170)；
      | 第二帧头错=(Position==1) AND (Byte!=85)。
      |
      | 例：Position=1、Byte=AA时，字节是AA和第二帧头错都为真。这并不冲突：它表示没等到55，但可以
      | 把这个AA视作重新找头的机会。是否写入、位置如何调整由后面两步分别处理。
      |
      | 本步骤不检查Active；本字节无效时，后面的写入和位置保持分支会阻止它改变状态。
  输入1_本项字节 : Inport
  输入2_本次之前已收字节数 : Inport  Port=2
  位置为0_等待AA : RelationalOperator  Operator===  OutDataTypeStr=boolean  RndMeth=Simplest  InputSameDT=off
  位置为1_等待55 : RelationalOperator  Operator===  OutDataTypeStr=boolean  RndMeth=Simplest  InputSameDT=off
  已见AA时位置1 : Constant  OutDataTypeStr=uint16
  帧头55_十进制85 : Constant  Value=85  OutDataTypeStr=uint8
  帧头AA_十进制170 : Constant  Value=170  OutDataTypeStr=uint8
  当前字节不是55 : RelationalOperator  Operator=~=  OutDataTypeStr=boolean  RndMeth=Simplest  InputSameDT=off
  当前字节是否AA : RelationalOperator  Operator===  OutDataTypeStr=boolean  RndMeth=Simplest  InputSameDT=off
  等待55却收到其他值 : Logic  IconShape=distinctive  AllPortsSameDT=off  OutDataTypeStr=boolean
  起始位置0 : Constant  Value=0  OutDataTypeStr=uint16
  输出1_当前字节等于AA : Outport
  输出2_正在寻找第一个AA : Outport  Port=2
  输出3_第二帧头不匹配 : Outport  Port=3
  wires:
  等待55却收到其他值/1 -> 输出3_第二帧头不匹配/1
  位置为0_等待AA/1 -> 输出2_正在寻找第一个AA/1
  当前字节是否AA/1 -> 输出1_当前字节等于AA/1
  起始位置0/1 -> 位置为0_等待AA/2
  已见AA时位置1/1 -> 位置为1_等待55/2
  输入2_本次之前已收字节数/1 -> 位置为1_等待55/1, 位置为0_等待AA/1
  帧头55_十进制85/1 -> 当前字节不是55/2
  帧头AA_十进制170/1 -> 当前字节是否AA/2
  输入1_本项字节/1 -> 当前字节是否AA/1, 当前字节不是55/1
  当前字节不是55/1 -> 等待55却收到其他值/2
  位置为1_等待55/1 -> 等待55却收到其他值/1

== system turbo_controller/BoardInput_输入换算与协议解析/In02_Motor（电机反馈解析）/Receive（逐字节组帧与保持有效结果）_235/Step02_拼帧并保存半帧/Collect（帧头识别与缓存推进）_167/Step02_判断本字节能否写入 ==
  note: 第二步：决定本字节是否允许写进帧缓存
      |
      | 收帧必须先找到头，所以不是每个字节都写。将第一步的三个判断与Active组合：
      |
      | 允许写入=Active AND [
      |   (正在等AA AND 字节是AA)
      |   OR (不在等AA AND 第二帧头没有错)
      | ]。
      |
      | 分别理解：
      | 还在找AA时，只写AA，其他噪声不进入缓存；
      | 已经见到AA、等待55时，只写正确的55；
      | 头部已经确认后，按顺序接收普通数据，不因数据恰好是AA/55就重新找头；
      | Active为假时，上述条件再合适也不写。
      |
      | 例：已见AA后又来AA，本步骤不把第二个AA写进第2项；后面的重同步位置逻辑仍保留“已见AA”的状
      | 态，继续等55。
      |
      | 输出只是一项布尔写许可，送第四步。它不产生新缓存，也不判断整帧校验。
  输入1_正在寻找第一个AA : Inport
  输入2_当前字节等于AA : Inport  Port=2
  输入3_第二帧头不匹配 : Inport  Port=3
  输入4_本项字节有效 : Inport  Port=4
  字节符合收帧规则 : Logic  Operator=OR  IconShape=distinctive  AllPortsSameDT=off  OutDataTypeStr=boolean
  已经越过寻找AA阶段 : Logic  Operator=NOT  Inputs=1  IconShape=distinctive  AllPortsSameDT=off  OutDataTypeStr=boolean
  已过起点且第二帧头没错 : Logic  IconShape=distinctive  AllPortsSameDT=off  OutDataTypeStr=boolean
  本字节有效且允许写入 : Logic  IconShape=distinctive  AllPortsSameDT=off  OutDataTypeStr=boolean
  第二帧头没有错 : Logic  Operator=NOT  Inputs=1  IconShape=distinctive  AllPortsSameDT=off  OutDataTypeStr=boolean
  起点遇到AA : Logic  IconShape=distinctive  AllPortsSameDT=off  OutDataTypeStr=boolean
  输出1_本字节允许写缓存 : Outport
  wires:
  本字节有效且允许写入/1 -> 输出1_本字节允许写缓存/1
  字节符合收帧规则/1 -> 本字节有效且允许写入/2
  输入4_本项字节有效/1 -> 本字节有效且允许写入/1
  输入3_第二帧头不匹配/1 -> 第二帧头没有错/1
  已过起点且第二帧头没错/1 -> 字节符合收帧规则/2
  起点遇到AA/1 -> 字节符合收帧规则/1
  第二帧头没有错/1 -> 已过起点且第二帧头没错/2
  已经越过寻找AA阶段/1 -> 已过起点且第二帧头没错/1
  输入2_当前字节等于AA/1 -> 起点遇到AA/2
  输入1_正在寻找第一个AA/1 -> 起点遇到AA/1, 已经越过寻找AA阶段/1

== system turbo_controller/BoardInput_输入换算与协议解析/In02_Motor（电机反馈解析）/Receive（逐字节组帧与保持有效结果）_235/Step02_拼帧并保存半帧/Collect（帧头识别与缓存推进）_167/Step03_计算写入位置与是否满帧 ==
  note: 第三步：算本次写到第几项，并判断是否到帧尾
      |
      | Position表示本次之前已接收多少项。本次候选写入位置=Position+1；帧长度固定为9，达到帧尾=(候
      | 选写入位置==9)。
      |
      | 例如Position=0时，候选位置是1，AA应写到第1项；Position=1时，55应写到第2项；Position=8时，
      | 本次候选位置是9，这是最后一项。
      |
      | 注意这里算的是“候选位置”：即使Active为假，仍可计算Position+1，但第四、第五步会保持缓存和
      | 位置。不能仅因候选位置等于9就认定收到新帧。
      |
      | 候选位置送第四步写缓存；它及“达到帧尾”标志也送第五步，决定继续推进还是收齐后回0。本处不
      | 保存Position，也不清空缓存。
  输入1_本次之前已收字节数 : Inport
  候选位置是否到帧尾 : RelationalOperator  Operator===  OutDataTypeStr=boolean  RndMeth=Simplest  InputSameDT=off
  固定帧长9 : Constant  Value=9  OutDataTypeStr=uint16
  本次候选位置加一 : Sum  SaturateOnIntegerOverflow=on  OutDataTypeStr=Inherit: Same as first input
  每次推进1项 : Constant  OutDataTypeStr=uint16
  输出1_候选位置达到帧长 : Outport
  输出2_候选写入位置 : Outport  Port=2
  wires:
  候选位置是否到帧尾/1 -> 输出1_候选位置达到帧长/1
  每次推进1项/1 -> 本次候选位置加一/2
  输入1_本次之前已收字节数/1 -> 本次候选位置加一/1
  固定帧长9/1 -> 候选位置是否到帧尾/2
  本次候选位置加一/1 -> 候选位置是否到帧尾/1, 输出2_候选写入位置/1
